simulink model "My_gfm_battery_sil"  (R2018b)
settings: Solver=ode45  StartTime=0.0  StopTime=100  MaxStep=1e-4  RelTol=1e-3
PreLoadFcn:
  | modelDir = fileparts(get_param(bdroot,'FileName'));
  | 
  | load_system(fullfile(modelDir,'controls_element_lib.slx'));
  | load_system(fullfile(modelDir,'test_sequence_lib.slx'));
InitFcn:
  | close all;
  | clear all;
  | clc;
  | 
  | % frequency nominals
  | F_NOM = 60;
  | W_NOM = 2 * pi * F_NOM;
  | 
  | % base values relative to inverter
  | % --------------------------------
  | VLL_INV_NOM = 480;
  | P_INV_NOM = 1e6;
  | Q_INV_NOM = 0.5e6;
  | S_INV_NOM = sqrt(P_INV_NOM^2 + Q_INV_NOM^2);
  | 
  | I_INV_BASE = S_INV_NOM/(sqrt(3)*VLL_INV_NOM);
  | Z_INV_BASE = VLL_INV_NOM^2/S_INV_NOM;
  | L_INV_BASE = Z_INV_BASE / W_NOM;
  | C_INV_BASE = 1 / (Z_INV_BASE * W_NOM);
  | 
  | % nominal ratings for power system model
  | % --------------------------------------
  | INVERTER_COUNT = 100;
  | 
  | VLV_NOM = VLL_INV_NOM;
  | VMV_NOM = 35e3;
  | VHV_NOM = 230e3;
  | S_PLANT = INVERTER_COUNT * S_INV_NOM;
  | 
  | N_GSU = VHV_NOM/VMV_NOM;
  | N_MVT = VMV_NOM/VLV_NOM;
  | 
  | I_LV_BASE = S_PLANT/(sqrt(3)*VLV_NOM);
  | I_MV_BASE = S_PLANT/(sqrt(3)*VMV_NOM);
  | I_HV_BASE = S_PLANT/(sqrt(3)*VHV_NOM);
  | 
  | Z_LV_BASE = VLV_NOM^2/S_PLANT;
  | Z_MV_BASE = VMV_NOM^2/S_PLANT;
  | Z_HV_BASE = VHV_NOM^2/S_PLANT;
  | 
  | L_LV_BASE = Z_LV_BASE / W_NOM;
  | L_MV_BASE = Z_MV_BASE / W_NOM;
  | L_HV_BASE = Z_HV_BASE / W_NOM;
  | C_LV_BASE = 1 / (Z_LV_BASE * W_NOM);
  | C_MV_BASE = 1 / (Z_MV_BASE * W_NOM);
  | C_HV_BASE = 1 / (Z_HV_BASE * W_NOM);
undefined symbols (not defined in the file): FreqFF_Sel, j
libraries: simulink x80, controls_element_lib x20, test_sequence_lib x16
(part 1 of 5)
settings Model: SimulationMode=accelerator  Creator=HussamAlatrash  LastModifiedBy=ahhei
settings DataIOCC: ReturnWorkspaceOutputs=on
settings OptimizationCC: EfficientMapNaN2IntZero=off
settings DebuggingCC: UnconnectedInputMsg=none  UnconnectedOutputMsg=none  UnconnectedLineMsg=none
settings HardwareCC: TargetBitPerPointer=64  TargetBitPerSizeT=64  TargetBitPerPtrDiffT=64  TargetLongLongMode=on  TargetIntDivRoundTo=Zero  TargetEndianess=LittleEndian  TargetWordSize=64  TargetHWDeviceType=MATLAB Host  ProdEqTarget=off
settings ModelReferenceCC: EnableRefExpFcnMdlSchedulingChecks=off
settings CodeAppCC: MaxIdLength=128
settings GRTTargetCC: TargetLangStandard=C89/C90 (ANSI)  CombineOutputUpdateFcns=off  GRTInterface=on

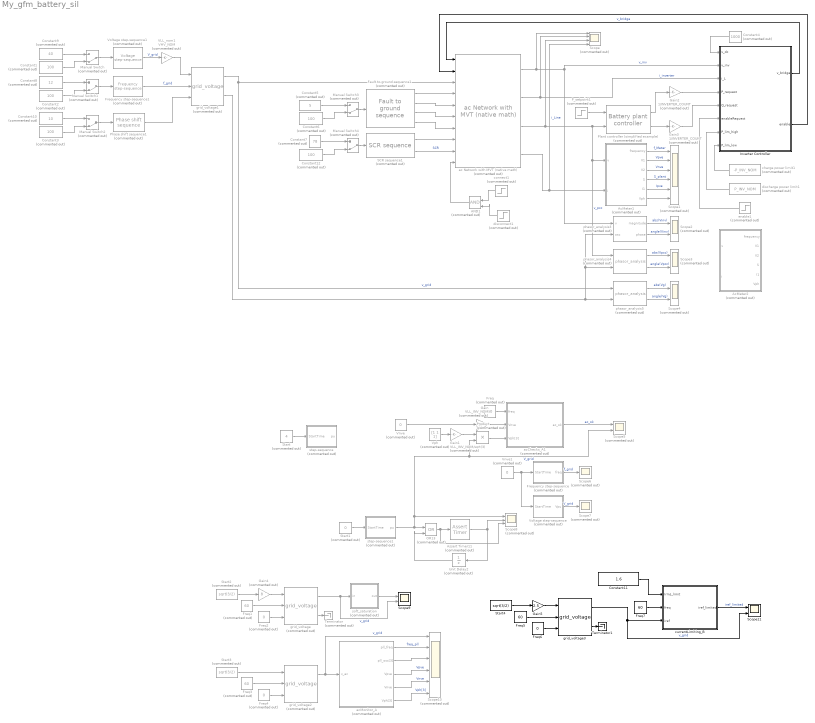
== system My_gfm_battery_sil ==
  AND1 : Logic  Commented=on  IconShape=distinctive  AllPortsSameDT=off  OutDataTypeStr=boolean
  AcMeter1 : Subsystem  Commented=on  AncestorBlock=test_sequence_lib/AcMeter  mask{VllRated=VHV_NOM}
      mask prompts: VllRated "Rated line voltage"
  AcMeter2 : Subsystem  Commented=on  AncestorBlock=test_sequence_lib/AcMeter  mask{VllRated=VHV_NOM}
      mask prompts: VllRated "Rated line voltage"
  Assert Timer11 : controls_element_lib/acChecks_A/Assert Timer  Commented=on  T_STEP=1e-3  TIMEOUT=2
  Constant{1..3,6,12} (5 alike) : Constant  Commented=on  Value=100
  Constant10 : Constant  Commented=on  Value=10
  Constant11 : Constant  Value=1.6
  Constant4 : Constant  Commented=on  Value=1000
  Constant5 : Constant  Commented=on  Value=5
  Constant7 : Constant  Commented=on  Value=78
  Constant8 : Constant  Commented=on  Value=12
  Constant9 : Constant  Commented=on  Value=40
  Fault to ground sequence1 : test_sequence_lib/Fault to ground sequence  Commented=on  SystemSampleTime=-1
  Freq : Constant  Commented=on  Value=60
  Freq1 : Constant  Commented=on  Value=60
  Freq2 : Constant  Commented=on  Value=0
  Freq3 : Constant  Commented=on  Value=60
  Freq4 : Constant  Commented=on  Value=0
  Freq5 : Constant  Value=60
  Freq6 : Constant  Value=0
  Freq7 : Constant  Value=60
  Frequency step-sequence : Subsystem  Commented=on  AncestorBlock=test_sequence_lib/Frequency step-sequence
  Frequency step-sequence1 : test_sequence_lib/Frequency step-sequence  Commented=on  SystemSampleTime=-1
  Gain : Gain  Commented=on  Gain=VLL_INV_NOM
  Gain1 : Gain  Commented=on  Gain=VLL_INV_NOM/sqrt(3)
  Gain2 : Gain  Commented=on  Gain=1/INVERTER_COUNT
  Gain3 : Gain  Commented=on  Gain=1/INVERTER_COUNT
  Gain4 : Gain  Commented=on  Gain=8
  Gain5 : Gain  Gain=2.5
  Inverter Controller : Subsystem
  Manual Switch{,1..4} (5 alike) : ManualSwitch  Commented=on  CurrentSetting=0
  OR13 : Logic  Commented=on  Operator=OR  IconShape=distinctive  AllPortsSameDT=off  OutDataTypeStr=boolean
  P_setpoint1 : Step  Commented=on  Time=4  After=S_PLANT*0.5  SampleTime=0
  Phase shift sequence1 : test_sequence_lib/Phase shift sequence  Commented=on  SystemSampleTime=-1
  Plant controller (simplified example) : controls_element_lib/Battery plant controller  Commented=on  SystemSampleTime=-1
  Product : Product  Commented=on
  SCR sequence1 : test_sequence_lib/SCR sequence  Commented=on  SystemSampleTime=-1
  Scope : Scope  Commented=on  NumInputPorts=4
  Scope1 : Scope  Commented=on  NumInputPorts=6
  Scope10 : Scope  Commented=on  NumInputPorts=6
  Scope11 : Scope  NumInputPorts=2
  Scope{2..5} (4 alike) : Scope  Commented=on  NumInputPorts=2
  Scope6 : Scope  Commented=on
  Scope7 : Scope  Commented=on
  Scope8 : Scope  Commented=on  NumInputPorts=3
  Scope9 : Scope  NumInputPorts=2
  Start : Constant  Commented=on  Value=4
  Start1 : Constant  Commented=on  Value=0
  Start2 : Constant  Commented=on  Value=sqrt(3/2)
  Start3 : Constant  Commented=on  Value=sqrt(3/2)
  Start4 : Constant  Value=sqrt(3/2)
  Terminator : Terminator  Commented=on
  Terminator1 : Terminator
  Unit Delay2 : UnitDelay  Commented=on  SampleTime=-1
  VLL_nom1 : Gain  Commented=on  Gain=VHV_NOM
  Vnve : Constant  Commented=on  Value=0
  Vnve1 : Constant  Commented=on  Value=0
  Voltage step-sequence : Subsystem  Commented=on  AncestorBlock=test_sequence_lib/Voltage step-sequence
  Voltage step-sequence1 : test_sequence_lib/Voltage step-sequence  Commented=on  SystemSampleTime=-1
  Vph : Constant  Commented=on  Value=[1 1 1]
  ac Network with MVT (native math) : test_sequence_lib/ac Network with MVT (native math)  Commented=on  SystemSampleTime=-1
  acChecks_A1 : Subsystem  Commented=on  AncestorBlock=controls_element_lib/acChecks_A  mask{VllRated=VLL_INV_NOM, nominalFrequency=F_NOM, tRequalify=2, T_CNTL=1e-3}
      mask prompts: VllRated "Rated line-to-line voltage (V)"; nominalFrequency "Nominal line frequency (Hz)"; tRequalify "Reconnection time (sec)"; T_CNTL "Operating sample time"
  "acMonitor_A " : Subsystem  Commented=on  AncestorBlock=controls_element_lib/acMonitor_A  mask{VllRated=VLL_INV_NOM, nominalFrequency=F_NOM}
      mask prompts: VllRated "Rated line-to-line voltage (V)"; nominalFrequency "Nominal line frequency (Hz)"
  charge power limit1 : Constant  Commented=on  Value=-P_INV_NOM
  connect1 : Step  Commented=on  Time=0  SampleTime=0
  currentLimiting_B : Subsystem  AncestorBlock=controls_element_lib/currentLimiting_B  mask{IRated=1, peakSoftLimit=2.6, peakHardLimit=3.6}
      mask prompts: IRated "Rated current (A)"; peakSoftLimit "Soft peak limit (pu)"; peakHardLimit "Hard peak limit (pu)"
  discharge power limit1 : Constant  Commented=on  Value=P_INV_NOM
  disconnect1 : Step  Commented=on  Time=10  Before=1  After=0  SampleTime=0
  enable1 : Step  Commented=on  Time=0.5  SampleTime=0
  grid_voltage : test_sequence_lib/grid_voltage  Commented=on  SystemSampleTime=-1
  grid_voltage1 : test_sequence_lib/grid_voltage  Commented=on  SystemSampleTime=-1
  grid_voltage2 : test_sequence_lib/grid_voltage  Commented=on  SystemSampleTime=-1
  grid_voltage3 : test_sequence_lib/grid_voltage  SystemSampleTime=-1
  phasor_analysis3 : Subsystem  Commented=on  AncestorBlock=test_sequence_lib/phasor_analysis
  phasor_analysis4 : test_sequence_lib/phasor_analysis  Commented=on  SystemSampleTime=-1
  phasor_analysis5 : test_sequence_lib/phasor_analysis  Commented=on  SystemSampleTime=-1
  soft_saturation : Subsystem  Commented=on  mask{soft_limit=2.6*sqrt(2)*sqrt(1/2), hard_limit=3.6*sqrt(2)*sqrt(1/2), Xau=1}
      mask prompts: soft_limit "Soft limit"; hard_limit "Hard limit"; Xau "Saturation Rate"
  step-sequence : Subsystem  Commented=on  AncestorBlock=test_sequence_lib/Voltage step-sequence
  step-sequence1 : Subsystem  Commented=on  AncestorBlock=test_sequence_lib/Voltage step-sequence
  wires:
  Voltage step-sequence1/1 -> VLL_nom1/1  "V_grid"
  Manual Switch/1 -> Voltage step-sequence1/1
  Fault to ground sequence1/2 -> ac Network with MVT (native math)/5
  AND1/1 -> ac Network with MVT (native math)/10
  Constant4/1 -> Inverter Controller/1(v_dc)
  AcMeter1/3(V2) -> Scope1/3  "Vnve"
  discharge power limit1/1 -> Inverter Controller/7(P_lim_high)
  Fault to ground sequence1/3 -> ac Network with MVT (native math)/6
  AcMeter1/6(Vph) -> Scope1/6
  Inverter Controller/1(v_bridge) -> ac Network with MVT (native math)/1  "v_bridge"
  AcMeter1/2(V1) -> Scope1/2  "Vpve"
  Plant controller (simplified example)/1 -> Gain2/1
  ac Network with MVT (native math)/1 -> Inverter Controller/2(v_inv), phasor_analysis3/1(v), Scope/1  "v_inv"
  P_setpoint1/1 -> Plant controller (simplified example)/1
  phasor_analysis5/1 -> Scope4/1  "abs(Vg)"
  AcMeter1/5(I1) -> Scope1/5  "Ipve"
  Gain3/1 -> Inverter Controller/5(Q_request)
  Plant controller (simplified example)/2 -> Gain3/1
  grid_voltage1/1 -> ac Network with MVT (native math)/3, phasor_analysis5/1  "v_grid"
  SCR sequence1/1 -> ac Network with MVT (native math)/8
  phasor_analysis3/1(magnitude) -> Scope2/1  "abs(Vinv)"
  Phase shift sequence1/1 -> grid_voltage1/3
  AcMeter1/4(S) -> Scope1/4  "S_plant"
  ac Network with MVT (native math)/4 -> Scope/4, AcMeter1/2(i)  "i_Line"
  AcMeter1/1(frequency) -> Scope1/1  "f_Meter"
  VLL_nom1/1 -> grid_voltage1/1
  phasor_analysis3/2(phase) -> Scope2/2  "angle(Vinv)"
  SCR sequence1/2 -> ac Network with MVT (native math)/9  "SCR"
  ac Network with MVT (native math)/2 -> Inverter Controller/3(i_L), Scope/2  "i_inverter"
  disconnect1/1 -> AND1/2
  Fault to ground sequence1/4 -> ac Network with MVT (native math)/7
  Gain2/1 -> Inverter Controller/4(P_request)
  ac Network with MVT (native math)/3 -> Plant controller (simplified example)/2, phasor_analysis4/1, AcMeter1/1(v), Scope/3  "v_pcc"
  charge power limit1/1 -> Inverter Controller/8(P_lim_low)
  Inverter Controller/2(enable) -> ac Network with MVT (native math)/2
  Frequency step-sequence1/1 -> grid_voltage1/2  "f_grid"
  Fault to ground sequence1/1 -> ac Network with MVT (native math)/4
  grid_voltage1/2 -> phasor_analysis4/2, phasor_analysis3/2(osc), phasor_analysis5/2
  phasor_analysis5/2 -> Scope4/2  "angle(Vg)"
  enable1/1 -> Inverter Controller/6(enableRequest)
  connect1/1 -> AND1/1
  Constant9/1 -> Manual Switch/1
  Constant1/1 -> Manual Switch/2
  Constant2/1 -> Manual Switch1/2
  Manual Switch1/1 -> Frequency step-sequence1/1
  Constant8/1 -> Manual Switch1/1
  Manual Switch2/1 -> Phase shift sequence1/1
  Constant3/1 -> Manual Switch2/2
  Constant10/1 -> Manual Switch2/1
  Constant6/1 -> Manual Switch3/2
  Constant5/1 -> Manual Switch3/1
  Manual Switch3/1 -> Fault to ground sequence1/1
  Constant7/1 -> Manual Switch4/1
  Constant12/1 -> Manual Switch4/2
  Manual Switch4/1 -> SCR sequence1/1
  phasor_analysis4/1 -> Scope3/1  "abs(Vpcc)"
  phasor_analysis4/2 -> Scope3/2  "angle(Vpcc)"
  Vnve/1 -> Gain/1
  Freq/1 -> acChecks_A1/1(freq)
  Vph/1 -> Gain1/1
  acChecks_A1/1(ac_ok) -> Scope5/1  "ac_ok"
  Gain/1 -> acChecks_A1/2(Vnve)
  Vnve1/1 -> Voltage step-sequence/1(StartTime), Frequency step-sequence/1(StartTime)
  Frequency step-sequence/1(freq) -> Scope6/1  "f_grid"
  Voltage step-sequence/1(Vpu) -> Scope7/1  "V_grid"
  Start/1 -> step-sequence/1(StartTime)
  Gain1/1 -> Product/1
  Product/1 -> acChecks_A1/3(Vph[3])
  step-sequence1/1(pu) -> Scope5/2, Product/2, Scope8/1, OR13/1  "V_grid"
  OR13/1 -> Scope8/3, Assert Timer11/1
  Unit Delay2/1 -> OR13/2
  Start1/1 -> step-sequence1/1(StartTime)
  Assert Timer11/1 -> Scope8/2, Unit Delay2/1
  grid_voltage/1 -> Scope9/2, soft_saturation/1(in)  "v_grid"
  Start2/1 -> Gain4/1
  Gain4/1 -> grid_voltage/1
  Freq1/1 -> grid_voltage/2
  Freq2/1 -> grid_voltage/3
  soft_saturation/1(out) -> Scope9/1
  grid_voltage/2 -> Terminator/1
  Freq4/1 -> grid_voltage2/3
  Freq3/1 -> grid_voltage2/2
  Start3/1 -> grid_voltage2/1
  grid_voltage2/1 -> Scope10/1, "acMonitor_A "/1(v_ac)  "v_grid"
  "acMonitor_A "/1(pll_freq) -> Scope10/2  "freq_pll"
  "acMonitor_A "/2(pll_osc[3]) -> Scope10/3
  "acMonitor_A "/3(Vpve) -> Scope10/4  "Vpve"
  "acMonitor_A "/4(Vnve) -> Scope10/5  "Vnve"
  "acMonitor_A "/5(Vph[3]) -> Scope10/6  "Vph[3]"
  Constant11/1 -> currentLimiting_B/1(Irms_limit)
  Start4/1 -> Gain5/1
  Freq6/1 -> grid_voltage3/3
  Gain5/1 -> grid_voltage3/1
  Freq5/1 -> grid_voltage3/2
  grid_voltage3/2 -> Terminator1/1
  grid_voltage3/1 -> Scope11/2, currentLimiting_B/3(iref)  "v_grid"
  Freq7/1 -> currentLimiting_B/2(freq)
  currentLimiting_B/1(iref_limited) -> Scope11/1  "iref_limited"

== system My_gfm_battery_sil/AcMeter1 ==
  v : Inport
  i : Inport  Port=2
  Conj : Math  Operator=conj  SaturateOnIntegerOverflow=on
  PLL_3ph : Subsystem
  Product : Product
  RMS calculator : Subsystem
  Scope : Scope  NumInputPorts=3
  Scope1 : Scope  NumInputPorts=4
  Sum of Elements : Sum  Commented=through  Inputs=+
  overVnom : Gain  Gain=1/VllRated
  phasor_analysis : Subsystem
  phasor_analysis1 : Subsystem  AncestorBlock=test_sequence_lib/AcMeter/phasor_analysis
  sqrt(3) : Gain  Gain=sqrt(3)
  sqrt(3)1 : Gain  Gain=sqrt(3)
  frequency : Outport  VectorParamsAs1DForOutWhenUnconnected=on
  V1 : Outport  Port=2  VectorParamsAs1DForOutWhenUnconnected=on
  V2 : Outport  Port=3  VectorParamsAs1DForOutWhenUnconnected=on
  S : Outport  Port=4  VectorParamsAs1DForOutWhenUnconnected=on
  I1 : Outport  Port=5  VectorParamsAs1DForOutWhenUnconnected=on
  Vph : Outport  Port=6  VectorParamsAs1DForOutWhenUnconnected=on
  wires:
  RMS calculator/1(out[3]) -> Vph/1
  PLL_3ph/2(osc[3]) -> phasor_analysis/2(osc), phasor_analysis1/2(osc)
  phasor_analysis/1(perPh) -> Scope/1
  Sum of Elements/1 -> Scope1/4, S/1  "S"
  v/1 -> RMS calculator/1(in[3]), phasor_analysis/1(in), overVnom/1
  PLL_3ph/1(freq) -> frequency/1
  overVnom/1 -> PLL_3ph/1(ref)
  Conj/1 -> Scope1/2, Product/2
  Product/1 -> Scope1/3, Sum of Elements/1
  phasor_analysis/2(pve) -> Scope/2, Scope1/1, Product/1, sqrt(3)/1  "Vpve_LN"
  phasor_analysis/3(nve) -> Scope/3, sqrt(3)1/1
  phasor_analysis1/2(pve) -> I1/1, Conj/1  "Ipve"
  sqrt(3)1/1 -> V2/1  "Vnve_LL"
  i/1 -> phasor_analysis1/1(in)
  sqrt(3)/1 -> V1/1  "Vpve_LL"

== system My_gfm_battery_sil/AcMeter2 ==
  v : Inport
  i : Inport  Port=2
  Conj : Math  Operator=conj  SaturateOnIntegerOverflow=on
  PLL_3ph : Subsystem
  Product : Product
  RMS calculator : Subsystem
  Scope : Scope  NumInputPorts=3
  Scope1 : Scope  NumInputPorts=4
  Sum of Elements : Sum  Inputs=+
  overVnom : Gain  Gain=1/VllRated
  phasor_analysis : Subsystem
  phasor_analysis1 : Subsystem  AncestorBlock=test_sequence_lib/AcMeter/phasor_analysis
  sqrt(3) : Gain  Gain=sqrt(3)
  sqrt(3)1 : Gain  Gain=sqrt(3)
  frequency : Outport  VectorParamsAs1DForOutWhenUnconnected=on
  V1 : Outport  Port=2  VectorParamsAs1DForOutWhenUnconnected=on
  V2 : Outport  Port=3  VectorParamsAs1DForOutWhenUnconnected=on
  S : Outport  Port=4  VectorParamsAs1DForOutWhenUnconnected=on
  I1 : Outport  Port=5  VectorParamsAs1DForOutWhenUnconnected=on
  Vph : Outport  Port=6  VectorParamsAs1DForOutWhenUnconnected=on
  wires:
  RMS calculator/1(out[3]) -> Vph/1
  PLL_3ph/2(osc[3]) -> phasor_analysis/2(osc), phasor_analysis1/2(osc)
  phasor_analysis/1(perPh) -> Scope/1, Product/1, Scope1/1
  Sum of Elements/1 -> Scope1/4, S/1  "S"
  v/1 -> RMS calculator/1(in[3]), phasor_analysis/1(in), overVnom/1
  PLL_3ph/1(freq) -> frequency/1
  phasor_analysis1/1(perPh) -> Conj/1
  overVnom/1 -> PLL_3ph/1(ref)
  Conj/1 -> Scope1/2, Product/2
  Product/1 -> Scope1/3, Sum of Elements/1
  phasor_analysis/2(pve) -> Scope/2, sqrt(3)/1  "Vpve_LN"
  phasor_analysis/3(nve) -> Scope/3, sqrt(3)1/1
  phasor_analysis1/2(pve) -> I1/1  "Ipve"
  sqrt(3)1/1 -> V2/1  "Vnve_LL"
  i/1 -> phasor_analysis1/1(in)
  sqrt(3)/1 -> V1/1  "Vpve_LL"

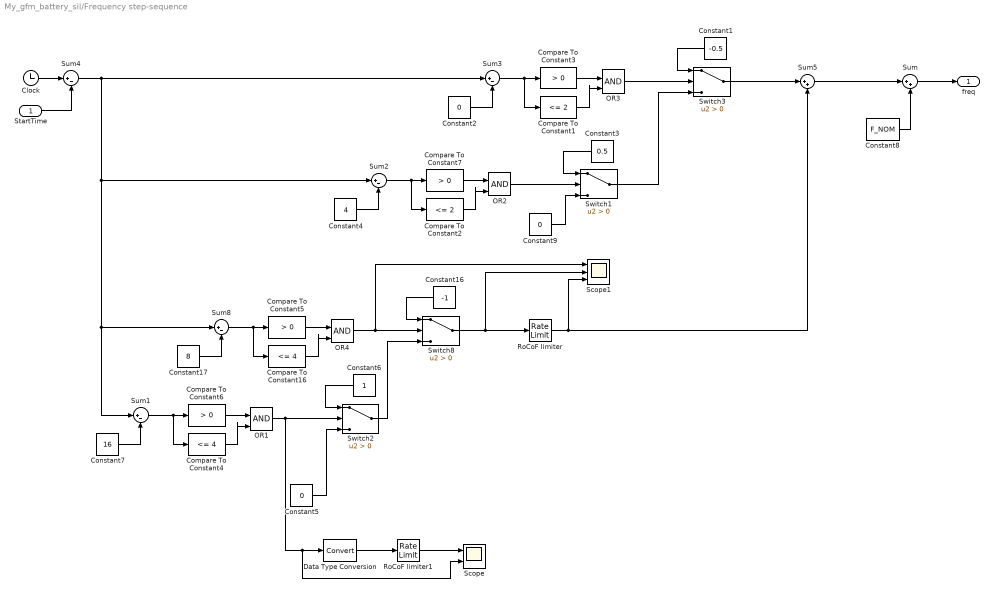
== system My_gfm_battery_sil/Frequency step-sequence ==
  StartTime : Inport
  Clock : Clock
  Compare To Constant1 : simulink/Logic and Bit Operations/Compare To Constant  relop=<=  const=2  OutDataTypeStr=boolean
  Compare To Constant16 : simulink/Logic and Bit Operations/Compare To Constant  relop=<=  const=4  OutDataTypeStr=boolean
  Compare To Constant2 : simulink/Logic and Bit Operations/Compare To Constant  relop=<=  const=2  OutDataTypeStr=boolean
  Compare To Constant{3,5..7} (4 alike) : simulink/Logic and Bit Operations/Compare To Constant  relop=>  const=0  OutDataTypeStr=boolean
  Compare To Constant4 : simulink/Logic and Bit Operations/Compare To Constant  relop=<=  const=4  OutDataTypeStr=boolean
  Constant1 : Constant  Value=-0.5
  Constant16 : Constant  Value=-1
  Constant17 : Constant  Value=8
  Constant2 : Constant  Value=0
  Constant3 : Constant  Value=0.5
  Constant4 : Constant  Value=4
  Constant5 : Constant  Value=0
  Constant6 : Constant
  Constant7 : Constant  Value=16
  Constant8 : Constant  Value=F_NOM
  Constant9 : Constant  Value=0
  Data Type Conversion : DataTypeConversion
  OR{1..4} (4 alike) : Logic  IconShape=distinctive  AllPortsSameDT=off  OutDataTypeStr=boolean
  RoCoF limiter : RateLimiter  SampleTimeMode=inherited
  RoCoF limiter1 : RateLimiter  SampleTimeMode=inherited
  Scope : Scope  NumInputPorts=2
  Scope1 : Scope  NumInputPorts=3
  Sum : Sum  Inputs=|++
  Sum{1..4,8} (5 alike) : Sum  Inputs=|+-
  Sum5 : Sum  Inputs=|++
  Switch{1..3,8} (4 alike) : Switch  Criteria=u2 > Threshold
  freq : Outport  VectorParamsAs1DForOutWhenUnconnected=on
  wires:
  Switch2/1 -> Switch8/3
  Constant16/1 -> Switch8/1
  OR4/1 -> Scope1/1, Switch8/2
  Compare To Constant5/1 -> OR4/1
  Sum8/1 -> Compare To Constant5/1, Compare To Constant16/1
  Constant17/1 -> Sum8/2
  Compare To Constant16/1 -> OR4/2
  Constant5/1 -> Switch2/3
  Constant6/1 -> Switch2/1
  OR1/1 -> Scope/2, Data Type Conversion/1, Switch2/2
  Compare To Constant6/1 -> OR1/1
  Sum1/1 -> Compare To Constant6/1, Compare To Constant4/1
  Constant7/1 -> Sum1/2
  Compare To Constant4/1 -> OR1/2
  Compare To Constant2/1 -> OR2/2
  Constant4/1 -> Sum2/2
  Sum2/1 -> Compare To Constant2/1, Compare To Constant7/1
  Compare To Constant7/1 -> OR2/1
  OR2/1 -> Switch1/2
  Constant3/1 -> Switch1/1
  Compare To Constant1/1 -> OR3/2
  Constant2/1 -> Sum3/2
  Sum3/1 -> Compare To Constant1/1, Compare To Constant3/1
  Compare To Constant3/1 -> OR3/1
  OR3/1 -> Switch3/2
  Constant1/1 -> Switch3/1
  Sum4/1 -> Sum3/1, Sum2/1, Sum8/1, Sum1/1
  Switch1/1 -> Switch3/3
  Clock/1 -> Sum4/1
  StartTime/1 -> Sum4/2
  Switch8/1 -> Scope1/2, RoCoF limiter/1
  Sum/1 -> freq/1
  Constant8/1 -> Sum/2
  Sum5/1 -> Sum/1
  RoCoF limiter/1 -> Scope1/3, Sum5/2
  Constant9/1 -> Switch1/3
  RoCoF limiter1/1 -> Scope/1
  Data Type Conversion/1 -> RoCoF limiter1/1
  Switch3/1 -> Sum5/1

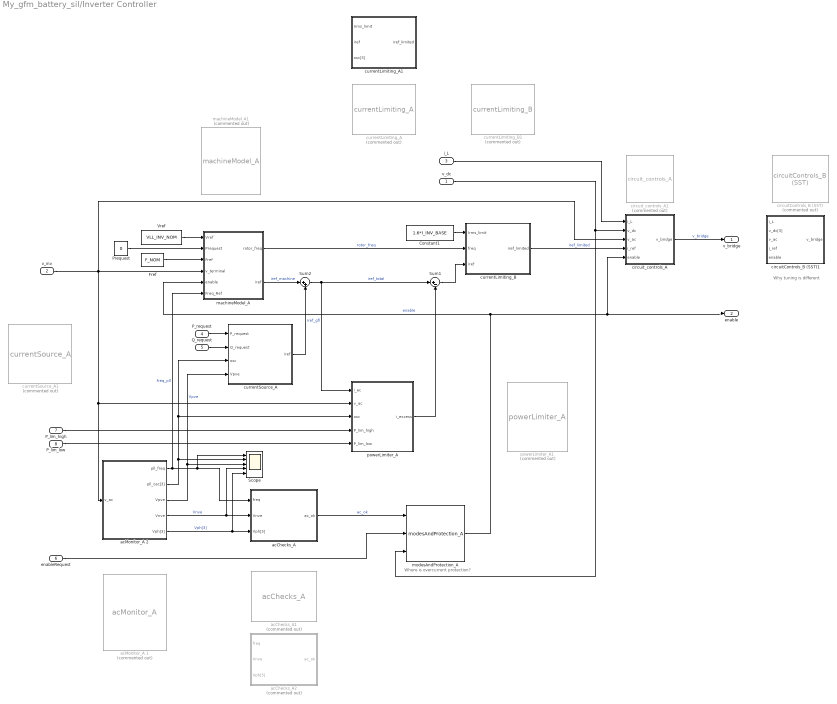
== system My_gfm_battery_sil/Inverter Controller ==
  note: Why tuning is different
  note: Where is overcurrent protection?
  v_dc : Inport
  v_inv : Inport  Port=2
  i_L : Inport  Port=3
  P_request : Inport  Port=4
  Q_request : Inport  Port=5
  enableRequest : Inport  Port=6
  P_lim_high : Inport  Port=7
  P_lim_low : Inport  Port=8
  Constant1 : Constant  Value=1.6*I_INV_BASE
  Fref : Constant  Value=F_NOM
  Prequest : Constant  Value=0
  Scope : Scope  NumInputPorts=5
  Sum1 : Sum  Inputs=|+-
  Sum2 : Sum  Inputs=|++
  Vref : Constant  Value=VLL_INV_NOM
  acChecks_A : Subsystem  AncestorBlock=controls_element_lib/acChecks_A  mask{VllRated=VLL_INV_NOM, nominalFrequency=F_NOM, tRequalify=2, T_CNTL=1e-3}
      mask prompts: VllRated "Rated line-to-line voltage (V)"; nominalFrequency "Nominal line frequency (Hz)"; tRequalify "Reconnection time (sec)"; T_CNTL "Operating sample time"
  acChecks_A1 : controls_element_lib/acChecks_A  Commented=on  VllRated=VLL_INV_NOM  nominalFrequency=F_NOM  tRequalify=2  T_CNTL=1e-3
  acChecks_A2 : Subsystem  Commented=on  AncestorBlock=controls_element_lib/acChecks_A  mask{VllRated=VLL_INV_NOM, NominalFrequency=F_NOM, Ts=1e-3, Time1=2, Time2=0, VHi=0, VLo=0, FHi=0, FLo=0, VNeg=0, Time3=0, OV1=0, OV1_Time=0, OV2=0, OV2_Time=0, OV3=0, OV3_Time=0, UV1=0, UV1_Time=0, UV2=0, UV2_Time=0, UV3=0, UV3_Time=0, OF1=0, OF1_Time=0, OF2=0, OF2_Time=0, OF3=0, OF3_Time=0, UF1=0, UF1_Time=0, UF2=0, UF2_Time=0, UF3=0, UF3_Time=0}
      mask prompts: VllRated "Rated Line-to-Line Voltage (V)"; NominalFrequency "Nominal Line Frequency (Hz)"; Ts "Operating Sample Time (sec)"; Time1 "Reconnection Time (sec)"; Time2 "Connect Out-of-Condition Delay (sec)"; VHi "High Voltage Threshold (pu)"; VLo "Low Voltage Threshold (pu)"; FHi "High Frequency Threshold (Hz)"; FLo "Low Frequency Threshold (Hz)"; VNeg "Negative Sequence Voltage Threshold (pu)"; Time3 "Trip Out-of-Condition Delay (sec)"; OV1 "OV PickUp 1 (pu)"; OV1_Time "OV Time 1 (sec)"; OV2 "OV PickUp 2 (pu)"; OV2_Time "OV Time 2 (sec)"; OV3 "OV PickUp 3 (pu)"; OV3_Time "OV Time 3 (sec)"; UV1 "UV PickUp 1 (pu)"; UV1_Time "UV Time 1 (sec)"; UV2 "UV PickUp 2 (pu)"; UV2_Time "UV Time 2 (sec)"; UV3 "UV PickUp 3 (pu)"; UV3_Time "UV Time 3 (sec)"; OF1 "OF PickUp 1 (Hz)"; OF1_Time "OF Time 1 (pu)"; OF2 "OF PickUp 2 (Hz)"; OF2_Time "OF Time 2 (pu)"; OF3 "OF PickUp 3 (Hz)"; OF3_Time "OF Time 3 (pu)"; UF1 "UF PickUp 1 (Hz)"; UF1_Time "UF Time 1 (sec)"; UF2 "UF PickUp 2 (Hz)"; UF2_Time "UF Time 2 (sec)"; UF3 "UF PickUp 3 (Hz)"; UF3_Time "UF Time 3 (sec)"
      mask DialogControl DescGroupVar Prompt: ACChecks
      mask DialogControl DecsTextVar Prompt: Grid Checks for Connection and Tripping
      mask DialogControl ParameterGroupVar Prompt: General Parameters
      mask DialogControl Container11 Prompt: Connect Settings
      mask DialogControl Container20 Prompt: Thresholds
      mask DialogControl Container3 Prompt: Trip Settings
      mask DialogControl Container12 Prompt: General Parameters
      mask DialogControl Container15 Prompt: Over Voltage Settings
      mask DialogControl Container4 Prompt: Over Voltage
      mask DialogControl Container19 Prompt: Under Voltage Settings
      mask DialogControl Container7 Prompt: Under Voltage
      mask DialogControl Container17 Prompt: Over Frequency Settings
      mask DialogControl Container9 Prompt: Over Frequency
      mask DialogControl Container16 Prompt: Under Frequency Settings
      mask DialogControl Container10 Prompt: Under Frequency
  acMonitor_A 1 : controls_element_lib/acMonitor_A  Commented=on  VllRated=VLL_INV_NOM  nominalFrequency=F_NOM
  acMonitor_A 2 : Subsystem  AncestorBlock=controls_element_lib/acMonitor_A  mask{VllRated=VLL_INV_NOM, nominalFrequency=F_NOM}
      mask prompts: VllRated "Rated line-to-line voltage (V)"; nominalFrequency "Nominal line frequency (Hz)"
  circuitControls_B (SST) : controls_element_lib/circuitControls_B (SST)  Commented=on  SystemSampleTime=-1
  circuitControls_B (SST)1 : Subsystem  AncestorBlock=controls_element_lib/circuitControls_B (SST)
  circuit_controls_A : Subsystem  AncestorBlock=controls_element_lib/circuit_controls_A
  circuit_controls_A1 : controls_element_lib/circuit_controls_A  Commented=on  SystemSampleTime=-1
  currentLimiting_A : controls_element_lib/currentLimiting_A  Commented=on  IRated=I_INV_BASE  peakSoftLimit=2.6  peakHardLimit=3.6
  currentLimiting_A1 : Subsystem  AncestorBlock=controls_element_lib/currentLimiting_A  mask{IRated=I_INV_BASE, peakSoftLimit=2.6, peakHardLimit=3.6}
      mask prompts: IRated "Rated current (A)"; peakSoftLimit "Soft peak limit (pu)"; peakHardLimit "Hard peak limit (pu)"
  currentLimiting_B : Subsystem  AncestorBlock=controls_element_lib/currentLimiting_B  mask{IRated=1, peakSoftLimit=2.6, peakHardLimit=3.6}
      mask prompts: IRated "Rated current (A)"; peakSoftLimit "Soft peak limit (pu)"; peakHardLimit "Hard peak limit (pu)"
  currentLimiting_B1 : controls_element_lib/currentLimiting_B  Commented=on  IRated=I_INV_BASE  peakSoftLimit=2.6  peakHardLimit=3.6
  currentSource_A : Subsystem  AncestorBlock=controls_element_lib/currentSource_A  mask{VllRated=VLL_INV_NOM, SRated=S_INV_NOM, nominalFrequency=F_NOM, Plimit=P_INV_NOM/S_INV_NOM, Qlimit=Q_INV_NOM/S_INV_NOM}
      mask prompts: VllRated "Rated line-to-line voltage (V)"; SRated "Rated power (VA)"; nominalFrequency "Nominal line frequency (Hz)"; Plimit "Real power request limit (pu)"; Qlimit "Reactive power request limit (pu)"
  currentSource_A1 : controls_element_lib/currentSource_A  Commented=on  VllRated=VLL_INV_NOM  SRated=S_INV_NOM  nominalFrequency=F_NOM  Plimit=P_INV_NOM/S_INV_NOM  Qlimit=Q_INV_NOM/S_INV_NOM
  machineModel_A : Subsystem  AncestorBlock=controls_element_lib/machineModel_A  mask{SRated=S_INV_NOM, VllRated=VLL_INV_NOM, nominalFrequency=F_NOM, inertialConstant=2.5, kDroop=1, kDamper=2, Xs=0.3, rs=0.08, Qlimit=0.5, wExciter=10}
      mask prompts: SRated "Rated power (VA)"; VllRated "Rated Voltage (Volts, line-to-line)"; nominalFrequency "Nominal frequency (Hz)"; inertialConstant "Inertial constant (seconds)"; kDroop "Droop gain (pu/Hz)"; kDamper "Damper gain (pu/Hz)"; Xs "Stator reactance (pu)"; rs "Stator resistance (pu)"; Qlimit "Reactive power request limit (pu)"; wExciter "Exciter Bandwidth (rad)"
  machineModel_A1 : controls_element_lib/machineModel_A  Commented=on  SRated=S_INV_NOM  VllRated=VLL_INV_NOM  nominalFrequency=F_NOM  inertialConstant=2.5  kDroop=1  kDamper=2  Xs=0.3  rs=0.08  Qlimit=0.5  wExciter=10
  modesAndProtection_A : controls_element_lib/modesAndProtection_A  dcOvervotlageThreshold=1800  dcUndervotlageThreshold=700  dcTripClearTimeout=0.2
  powerLimiter_A : Subsystem  AncestorBlock=controls_element_lib/powerLimiter_A  mask{VllRated=VLL_INV_NOM, nominalFrequency=F_NOM, wPowerLimiter=3}
      mask prompts: VllRated "Rated line-to-line voltage (V)"; nominalFrequency "Nominal line frequency (Hz)"; wPowerLimiter "Bandwidth (rad)"
  powerLimiter_A1 : controls_element_lib/powerLimiter_A  Commented=on  VllRated=VLL_INV_NOM  nominalFrequency=F_NOM  wPowerLimiter=3
  v_bridge : Outport  VectorParamsAs1DForOutWhenUnconnected=on
  enable : Outport  Port=2  VectorParamsAs1DForOutWhenUnconnected=on
  wires:
  Vref/1 -> machineModel_A/1(Vref)
  Prequest/1 -> machineModel_A/2(Prequest)
  Fref/1 -> machineModel_A/3(Fref)
  machineModel_A/2(iref) -> Sum2/1  "iref_machine"
  acMonitor_A 2/2(pll_osc[3]) -> Scope/2, currentSource_A/3(osc), powerLimiter_A/3(osc)
  currentLimiting_B/1(iref_limited) -> circuit_controls_A/4(i_ref)  "iref_limited"
  currentSource_A/1(iref) -> Sum2/2  "iref_gfl"
  Sum2/1 -> Sum1/1, powerLimiter_A/1(i_ac)  "iref_total"
  acMonitor_A 2/3(Vpve) -> Scope/3, currentSource_A/4(Vpve)  "Vpve"
  Q_request/1 -> currentSource_A/2(Q_request)
  P_request/1 -> currentSource_A/1(P_request)
  enableRequest/1 -> modesAndProtection_A/2
  modesAndProtection_A/1 -> machineModel_A/5(enable), circuit_controls_A/5(enable), enable/1  "enable"
  acMonitor_A 2/5(Vph[3]) -> Scope/5, acChecks_A/3(Vph[3])  "Vph[3]"
  acChecks_A/1(ac_ok) -> modesAndProtection_A/1  "ac_ok"
  Constant1/1 -> currentLimiting_B/1(Irms_limit)
  acMonitor_A 2/1(pll_freq) -> Scope/1, acChecks_A/1(freq), machineModel_A/6(Freq_Ref)  "freq_pll"
  acMonitor_A 2/4(Vnve) -> Scope/4, acChecks_A/2(Vnve)  "Vnve"
  P_lim_low/1 -> powerLimiter_A/5(P_lim_low)
  P_lim_high/1 -> powerLimiter_A/4(P_lim_high)
  powerLimiter_A/1(i_excess) -> Sum1/2
  Sum1/1 -> currentLimiting_B/3(iref)
  v_dc/1 -> circuit_controls_A/2(v_dc), modesAndProtection_A/3
  circuit_controls_A/1(v_bridge) -> v_bridge/1  "v_bridge"
  machineModel_A/1(rotor_freq) -> currentLimiting_B/2(freq)  "rotor_freq"
  i_L/1 -> circuit_controls_A/1(i_L)
  v_inv/1 -> acMonitor_A 2/1(v_ac), powerLimiter_A/2(v_ac), machineModel_A/4(v_terminal), circuit_controls_A/3(v_ac)

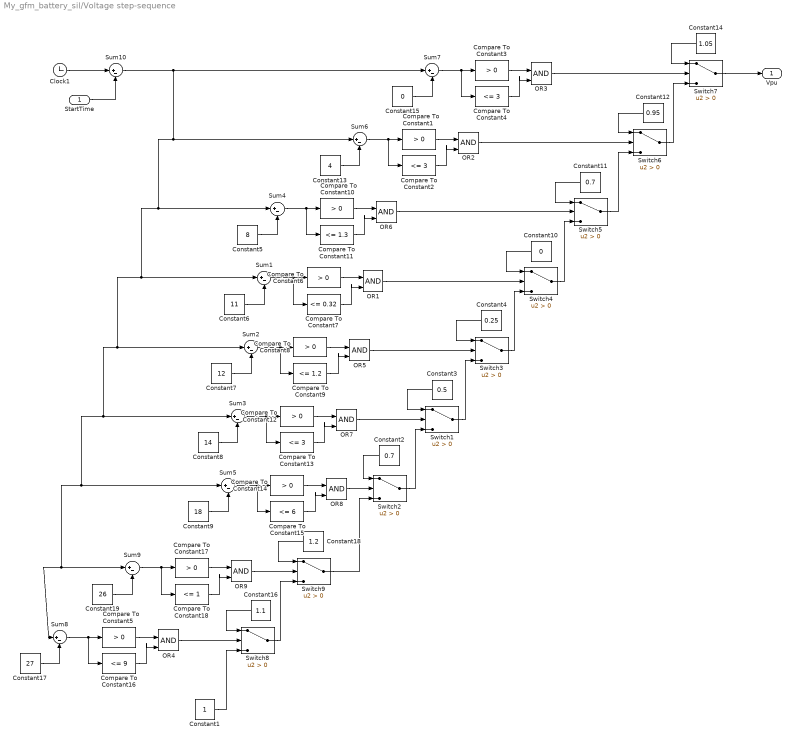
== system My_gfm_battery_sil/Voltage step-sequence ==
  StartTime : Inport
  Clock1 : Clock
  Compare To Constant{1,3,5..6,8,10,12,14,17} (9 alike) : simulink/Logic and Bit Operations/Compare To Constant  relop=>  const=0  OutDataTypeStr=boolean
  Compare To Constant11 : simulink/Logic and Bit Operations/Compare To Constant  relop=<=  const=1.3  OutDataTypeStr=boolean
  Compare To Constant13 : simulink/Logic and Bit Operations/Compare To Constant  relop=<=  const=3  OutDataTypeStr=boolean
  Compare To Constant15 : simulink/Logic and Bit Operations/Compare To Constant  relop=<=  const=6  OutDataTypeStr=boolean
  Compare To Constant16 : simulink/Logic and Bit Operations/Compare To Constant  relop=<=  const=9  OutDataTypeStr=boolean
  Compare To Constant18 : simulink/Logic and Bit Operations/Compare To Constant  relop=<=  const=1  OutDataTypeStr=boolean
  Compare To Constant2 : simulink/Logic and Bit Operations/Compare To Constant  relop=<=  const=3  OutDataTypeStr=boolean
  Compare To Constant4 : simulink/Logic and Bit Operations/Compare To Constant  relop=<=  const=3  OutDataTypeStr=boolean
  Compare To Constant7 : simulink/Logic and Bit Operations/Compare To Constant  relop=<=  const=0.32  OutDataTypeStr=boolean
  Compare To Constant9 : simulink/Logic and Bit Operations/Compare To Constant  relop=<=  const=1.2  OutDataTypeStr=boolean
  Constant1 : Constant
  Constant10 : Constant  Value=0
  Constant11 : Constant  Value=0.7
  Constant12 : Constant  Value=0.95
  Constant13 : Constant  Value=4
  Constant14 : Constant  Value=1.05
  Constant15 : Constant  Value=0
  Constant16 : Constant  Value=1.1
  Constant17 : Constant  Value=27
  Constant18 : Constant  Value=1.2
  Constant19 : Constant  Value=26
  Constant2 : Constant  Value=0.7
  Constant3 : Constant  Value=0.5
  Constant4 : Constant  Value=0.25
  Constant5 : Constant  Value=8
  Constant6 : Constant  Value=11
  Constant7 : Constant  Value=12
  Constant8 : Constant  Value=14
  Constant9 : Constant  Value=18
  OR{1..9} (9 alike) : Logic  IconShape=distinctive  AllPortsSameDT=off  OutDataTypeStr=boolean
  Sum{1..10} (10 alike) : Sum  Inputs=|+-
  Switch{1..9} (9 alike) : Switch  Criteria=u2 > Threshold
  Vpu : Outport  VectorParamsAs1DForOutWhenUnconnected=on
  wires:
  Constant2/1 -> Switch2/1
  Switch2/1 -> Switch1/3
  Switch9/1 -> Switch2/3
  OR7/1 -> Switch1/2
  Constant3/1 -> Switch1/1
  OR8/1 -> Switch2/2
  Sum4/1 -> Compare To Constant10/1, Compare To Constant11/1
  Constant5/1 -> Sum4/2
  OR6/1 -> Switch5/2
  Compare To Constant10/1 -> OR6/1
  Compare To Constant11/1 -> OR6/2
  Compare To Constant7/1 -> OR1/2
  Compare To Constant6/1 -> OR1/1
  Constant6/1 -> Sum1/2
  Sum1/1 -> Compare To Constant7/1, Compare To Constant6/1
  Sum2/1 -> Compare To Constant8/1, Compare To Constant9/1
  Constant7/1 -> Sum2/2
  Compare To Constant8/1 -> OR5/1
  Compare To Constant9/1 -> OR5/2
  Compare To Constant13/1 -> OR7/2
  Compare To Constant12/1 -> OR7/1
  Constant8/1 -> Sum3/2
  Sum3/1 -> Compare To Constant13/1, Compare To Constant12/1
  Sum5/1 -> Compare To Constant14/1, Compare To Constant15/1
  Constant9/1 -> Sum5/2
  Compare To Constant14/1 -> OR8/1
  Compare To Constant15/1 -> OR8/2
  Constant4/1 -> Switch3/1
  OR5/1 -> Switch3/2
  OR1/1 -> Switch4/2
  Constant10/1 -> Switch4/1
  Constant11/1 -> Switch5/1
  Switch1/1 -> Switch3/3
  Switch3/1 -> Switch4/3
  Switch4/1 -> Switch5/3
  Switch5/1 -> Switch6/3
  Constant12/1 -> Switch6/1
  Compare To Constant2/1 -> OR2/2
  Compare To Constant1/1 -> OR2/1
  OR2/1 -> Switch6/2
  Constant13/1 -> Sum6/2
  Sum6/1 -> Compare To Constant2/1, Compare To Constant1/1
  Sum7/1 -> Compare To Constant3/1, Compare To Constant4/1
  Constant15/1 -> Sum7/2
  OR3/1 -> Switch7/2
  Compare To Constant3/1 -> OR3/1
  Compare To Constant4/1 -> OR3/2
  Constant14/1 -> Switch7/1
  Switch6/1 -> Switch7/3
  Switch7/1 -> Vpu/1
  Switch8/1 -> Switch9/3
  Constant18/1 -> Switch9/1
  Sum10/1 -> Sum4/1, Sum1/1, Sum2/1, Sum3/1, Sum5/1, Sum8/1, Sum9/1, Sum6/1, Sum7/1
  Compare To Constant18/1 -> OR9/2
  Compare To Constant17/1 -> OR9/1
  OR9/1 -> Switch9/2
  Constant19/1 -> Sum9/2
  Sum9/1 -> Compare To Constant18/1, Compare To Constant17/1
  Sum8/1 -> Compare To Constant5/1, Compare To Constant16/1
  Constant17/1 -> Sum8/2
  OR4/1 -> Switch8/2
  Compare To Constant5/1 -> OR4/1
  Compare To Constant16/1 -> OR4/2
  Constant16/1 -> Switch8/1
  Constant1/1 -> Switch8/3
  Clock1/1 -> Sum10/1
  StartTime/1 -> Sum10/2

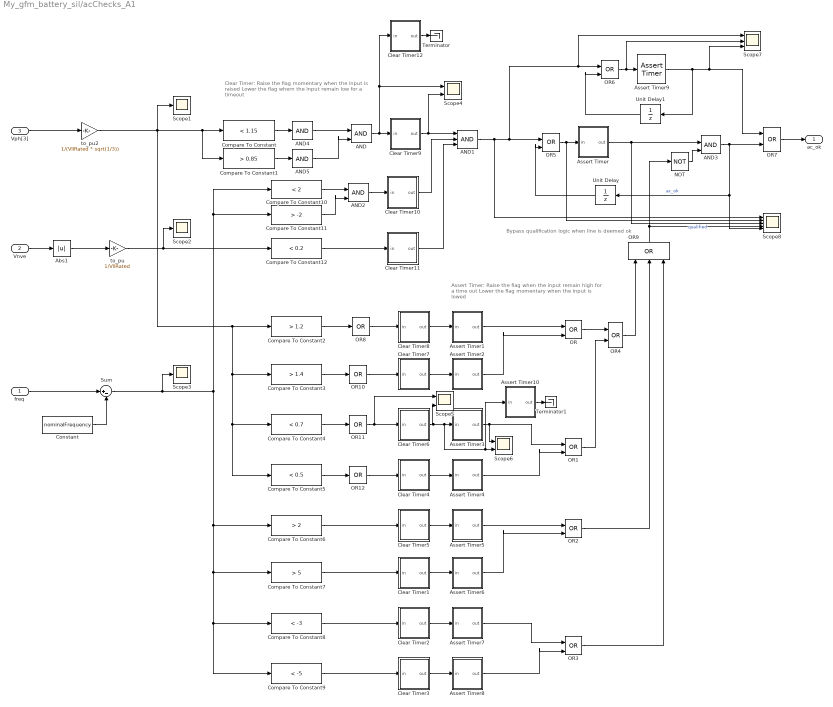
== system My_gfm_battery_sil/acChecks_A1 ==
  note: Clear Timer:
      | Raise the flag momentary when the input is raised
      | Lower the flag whern the input remain low for a timeout
  note: Bypass qualification logic when line is deemed ok
  note: Assert Timer:
      | Raise the flag when the input remain high for a time out
      | Lower the flag momentary when the input is lowed
  freq : Inport
  Vnve : Inport  Port=2
  Vph[3] : Inport  Port=3
  AND : Logic  IconShape=distinctive  AllPortsSameDT=off  OutDataTypeStr=boolean
  AND1 : Logic  Inputs=3  IconShape=distinctive  AllPortsSameDT=off  OutDataTypeStr=boolean
  AND2 : Logic  IconShape=distinctive  AllPortsSameDT=off  OutDataTypeStr=boolean
  AND3 : Logic  IconShape=distinctive  AllPortsSameDT=off  OutDataTypeStr=boolean
  AND4 : Logic  Inputs=1  IconShape=distinctive  AllPortsSameDT=off  OutDataTypeStr=boolean
  AND5 : Logic  Inputs=1  IconShape=distinctive  AllPortsSameDT=off  OutDataTypeStr=boolean
  Abs1 : Abs
  Assert Timer : Subsystem  mask{T_STEP=T_CNTL, TIMEOUT=300}
      mask prompts: T_STEP "Time step"
  Assert Timer1 : Subsystem  mask{T_STEP=T_CNTL, TIMEOUT=60}
      mask prompts: T_STEP "Time step"
  Assert Timer10 : Subsystem  mask{T_STEP=T_CNTL, TIMEOUT=60}
      mask prompts: T_STEP "Time step"
  Assert Timer2 : Subsystem  mask{T_STEP=T_CNTL, TIMEOUT=10}
      mask prompts: T_STEP "Time step"
  Assert Timer3 : Subsystem  mask{T_STEP=T_CNTL, TIMEOUT=60}
      mask prompts: T_STEP "Time step"
  Assert Timer4 : Subsystem  mask{T_STEP=T_CNTL, TIMEOUT=10}
      mask prompts: T_STEP "Time step"
  Assert Timer5 : Subsystem  mask{T_STEP=T_CNTL, TIMEOUT=60}
      mask prompts: T_STEP "Time step"
  Assert Timer6 : Subsystem  mask{T_STEP=T_CNTL, TIMEOUT=10}
      mask prompts: T_STEP "Time step"
  Assert Timer7 : Subsystem  mask{T_STEP=T_CNTL, TIMEOUT=60}
      mask prompts: T_STEP "Time step"
  Assert Timer8 : Subsystem  mask{T_STEP=T_CNTL, TIMEOUT=10}
      mask prompts: T_STEP "Time step"
  Assert Timer9 : controls_element_lib/acChecks_A/Assert Timer  T_STEP=T_CNTL  TIMEOUT=tRequalify
  Clear Timer1 : Subsystem  mask{T_STEP=T_CNTL, TIMEOUT=0.1, TIMER_INIT=0.1}
      mask prompts: T_STEP "Time step"; TIMER_INIT "Timer initial value"
  Clear Timer10 : Subsystem  mask{T_STEP=T_CNTL, TIMEOUT=0.1, TIMER_INIT=0}
      mask prompts: T_STEP "Time step"; TIMER_INIT "Timer initial value"
  Clear Timer11 : Subsystem  mask{T_STEP=T_CNTL, TIMEOUT=0.1, TIMER_INIT=0}
      mask prompts: T_STEP "Time step"; TIMER_INIT "Timer initial value"
  Clear Timer12 : Subsystem  mask{T_STEP=T_CNTL, TIMEOUT=0.1, TIMER_INIT=0}
      mask prompts: T_STEP "Time step"; TIMER_INIT "Timer initial value"
  Clear Timer2 : Subsystem  mask{T_STEP=T_CNTL, TIMEOUT=0.1, TIMER_INIT=0.1}
      mask prompts: T_STEP "Time step"; TIMER_INIT "Timer initial value"
  Clear Timer3 : Subsystem  mask{T_STEP=T_CNTL, TIMEOUT=0.1, TIMER_INIT=0.1}
      mask prompts: T_STEP "Time step"; TIMER_INIT "Timer initial value"
  Clear Timer4 : Subsystem  mask{T_STEP=T_CNTL, TIMEOUT=0.1, TIMER_INIT=0}
      mask prompts: T_STEP "Time step"; TIMER_INIT "Timer initial value"
  Clear Timer5 : Subsystem  mask{T_STEP=T_CNTL, TIMEOUT=0.1, TIMER_INIT=0.1}
      mask prompts: T_STEP "Time step"; TIMER_INIT "Timer initial value"
  Clear Timer6 : Subsystem  mask{T_STEP=T_CNTL, TIMEOUT=0.1, TIMER_INIT=0}
      mask prompts: T_STEP "Time step"; TIMER_INIT "Timer initial value"
  Clear Timer7 : Subsystem  mask{T_STEP=T_CNTL, TIMEOUT=0.1, TIMER_INIT=0}
      mask prompts: T_STEP "Time step"; TIMER_INIT "Timer initial value"
  Clear Timer8 : Subsystem  mask{T_STEP=T_CNTL, TIMEOUT=0.1, TIMER_INIT=0}
      mask prompts: T_STEP "Time step"; TIMER_INIT "Timer initial value"
  Clear Timer9 : Subsystem  mask{T_STEP=T_CNTL, TIMEOUT=0.1, TIMER_INIT=0}
      mask prompts: T_STEP "Time step"; TIMER_INIT "Timer initial value"
  Compare To Constant : simulink/Logic and Bit Operations/Compare To Constant  relop=<  const=1.15  OutDataTypeStr=boolean
  Compare To Constant1 : simulink/Logic and Bit Operations/Compare To Constant  relop=>  const=0.85  OutDataTypeStr=boolean
  Compare To Constant10 : simulink/Logic and Bit Operations/Compare To Constant  relop=<  const=2  OutDataTypeStr=boolean
  Compare To Constant11 : simulink/Logic and Bit Operations/Compare To Constant  relop=>  const=-2  OutDataTypeStr=boolean
  Compare To Constant12 : simulink/Logic and Bit Operations/Compare To Constant  relop=<  const=0.2  OutDataTypeStr=boolean
  Compare To Constant2 : simulink/Logic and Bit Operations/Compare To Constant  relop=>  const=1.2  OutDataTypeStr=boolean
  Compare To Constant3 : simulink/Logic and Bit Operations/Compare To Constant  relop=>  const=1.4  OutDataTypeStr=boolean
  Compare To Constant4 : simulink/Logic and Bit Operations/Compare To Constant  relop=<  const=0.7  OutDataTypeStr=boolean
  Compare To Constant5 : simulink/Logic and Bit Operations/Compare To Constant  relop=<  const=0.5  OutDataTypeStr=boolean
  Compare To Constant6 : simulink/Logic and Bit Operations/Compare To Constant  relop=>  const=2  OutDataTypeStr=boolean
  Compare To Constant7 : simulink/Logic and Bit Operations/Compare To Constant  relop=>  const=5  OutDataTypeStr=boolean
  Compare To Constant8 : simulink/Logic and Bit Operations/Compare To Constant  relop=<  const=-3  OutDataTypeStr=boolean
  Compare To Constant9 : simulink/Logic and Bit Operations/Compare To Constant  relop=<  const=-5  OutDataTypeStr=boolean
  Constant : Constant  Value=nominalFrequency
  NOT : Logic  Operator=NOT  IconShape=distinctive  AllPortsSameDT=off  OutDataTypeStr=boolean
  OR{,1..7} (8 alike) : Logic  Operator=OR  IconShape=distinctive  AllPortsSameDT=off  OutDataTypeStr=boolean
  OR{8,10..12} (4 alike) : Logic  Operator=OR  Inputs=1  IconShape=distinctive  AllPortsSameDT=off  OutDataTypeStr=boolean
  OR9 : Logic  Operator=OR  Inputs=3  IconShape=distinctive  AllPortsSameDT=off  OutDataTypeStr=boolean
  Scope1 : Scope
  Scope2 : Scope
  Scope3 : Scope
  Scope4 : Scope  NumInputPorts=2
  Scope5 : Scope  NumInputPorts=2
  Scope6 : Scope  NumInputPorts=2
  Scope7 : Scope  NumInputPorts=3
  Scope8 : Scope  NumInputPorts=5
  Sum : Sum  Inputs=|+-
  Terminator : Terminator
  Terminator1 : Terminator
  Unit Delay : UnitDelay  SampleTime=T_CNTL
  Unit Delay1 : UnitDelay  SampleTime=T_CNTL
  to_pu : Gain  Gain=1/VllRated
  to_pu2 : Gain  Gain=1/(VllRated * sqrt(1/3))
  ac_ok : Outport  VectorParamsAs1DForOutWhenUnconnected=on
  wires:
  Vph[3]/1 -> to_pu2/1
  OR4/1 -> OR9/1
  OR9/1 -> NOT/1, Scope8/4
  OR7/1 -> ac_ok/1
  Assert Timer9/1 -> Unit Delay1/1, Scope7/3, OR7/1
  OR6/1 -> Scope7/2, Assert Timer9/1
  Unit Delay1/1 -> OR6/2
  Constant/1 -> Sum/2
  freq/1 -> Sum/1
  to_pu/1 -> Scope2/1, Compare To Constant12/1
  to_pu2/1 -> Scope1/1, Compare To Constant/1, Compare To Constant1/1, Compare To Constant2/1, Compare To Constant5/1, Compare To Constant4/1, Compare To Constant3/1
  Abs1/1 -> to_pu/1
  Unit Delay/1 -> OR5/2
  Assert Timer1/1(out) -> OR/1
  Compare To Constant12/1 -> Clear Timer11/1(in)
  Clear Timer11/1(out) -> AND1/3
  Compare To Constant2/1 -> OR8/1
  Compare To Constant1/1 -> AND5/1
  Assert Timer/1(out) -> AND3/1, Scope8/3  "qualified"
  OR3/1 -> OR9/3
  Assert Timer4/1(out) -> OR1/2
  Assert Timer5/1(out) -> OR2/1
  Clear Timer5/1(out) -> Assert Timer5/1(in)
  Compare To Constant6/1 -> Clear Timer5/1(in)
  Clear Timer1/1(out) -> Assert Timer6/1(in)
  Clear Timer8/1(out) -> Assert Timer1/1(in)
  Assert Timer7/1(out) -> OR3/1
  Assert Timer8/1(out) -> OR3/2
  Vnve/1 -> Abs1/1
  NOT/1 -> AND3/2
  Assert Timer3/1(out) -> Scope6/1, OR1/1
  Compare To Constant/1 -> AND4/1
  Compare To Constant3/1 -> OR10/1
  AND2/1 -> Clear Timer10/1(in)
  Compare To Constant9/1 -> Clear Timer3/1(in)
  Compare To Constant11/1 -> AND2/2
  Compare To Constant4/1 -> OR11/1
  Assert Timer6/1(out) -> OR2/2
  Clear Timer6/1(out) -> Scope5/2, Assert Timer10/1(in), Scope6/2, Assert Timer3/1(in)
  Compare To Constant8/1 -> Clear Timer2/1(in)
  OR1/1 -> OR4/2
  Clear Timer2/1(out) -> Assert Timer7/1(in)
  Compare To Constant5/1 -> OR12/1
  Compare To Constant7/1 -> Clear Timer1/1(in)
  Clear Timer10/1(out) -> AND1/2
  Clear Timer3/1(out) -> Assert Timer8/1(in)
  Clear Timer7/1(out) -> Assert Timer2/1(in)
  Sum/1 -> Scope3/1, Compare To Constant11/1, Compare To Constant10/1, Compare To Constant6/1, Compare To Constant7/1, Compare To Constant8/1, Compare To Constant9/1
  Assert Timer2/1(out) -> OR/2
  Compare To Constant10/1 -> AND2/1
  Clear Timer9/1(out) -> Scope4/2, AND1/1
  OR/1 -> OR4/1
  Clear Timer4/1(out) -> Assert Timer4/1(in)
  AND3/1 -> Scope8/5, Unit Delay/1, OR7/2  "ac_ok"
  OR2/1 -> OR9/2
  OR8/1 -> Clear Timer8/1(in)
  OR10/1 -> Clear Timer7/1(in)
  OR11/1 -> Clear Timer6/1(in), Scope5/1
  OR12/1 -> Clear Timer4/1(in)
  AND/1 -> Clear Timer12/1(in), Scope4/1, Clear Timer9/1(in)
  AND4/1 -> AND/1
  AND5/1 -> AND/2
  Clear Timer12/1(out) -> Terminator/1
  Assert Timer10/1(out) -> Terminator1/1
  AND1/1 -> OR5/1, Scope7/1, OR6/1, Scope8/1
  OR5/1 -> Scope8/2, Assert Timer/1(in)

== system My_gfm_battery_sil/acMonitor_A  ==
  note: RMS LL Pos Seq Voltage (Vd+, Vq+)
  note: RMS LL Neg Seq Voltage (Vd-, Vq-)
  note: cos x + j sin x
      | cos (x-120) + j (sin x -120)
      | cos (x+120) + j (sin x +120)
  note: Hz
  note: RMS Va, Vb, Vc
  v_ac : Inport
  Analyzer_V : Subsystem
  Analyzer_V1 : Subsystem  Commented=on
  Gain2 : Gain  Gain=2
  PLL_3ph : Subsystem
  RMS_Analyzer : Subsystem
  SOGI : Subsystem
  Scope : Scope  NumInputPorts=3
  Scope1 : Scope  NumInputPorts=4
  Terminator : Terminator
  to_pu : Gain  Gain=1/VllRated
  pll_freq : Outport  VectorParamsAs1DForOutWhenUnconnected=on
  pll_osc[3] : Outport  Port=2  VectorParamsAs1DForOutWhenUnconnected=on
  Vpve : Outport  Port=3  VectorParamsAs1DForOutWhenUnconnected=on
  Vnve : Outport  Port=4  VectorParamsAs1DForOutWhenUnconnected=on
  Vph[3] : Outport  Port=5  VectorParamsAs1DForOutWhenUnconnected=on
  wires:
  SOGI/1(notch) -> Scope/3, Vph[3]/1
  Gain2/1 -> SOGI/2(fnom)
  RMS_Analyzer/1(RMS) -> Scope/2, SOGI/1(in)
  Analyzer_V/4(Nve) -> Scope1/4, Vnve/1
  Analyzer_V/3(Pve) -> Vpve/1, Scope1/3
  PLL_3ph/1(osc[3]) -> pll_osc[3]/1, Analyzer_V/2(osc[3])
  PLL_3ph/2(freq) -> Gain2/1, pll_freq/1
  v_ac/1 -> to_pu/1, Analyzer_V/1(in[3]), Scope/1, RMS_Analyzer/1(in)
  to_pu/1 -> PLL_3ph/1(ref)
  Analyzer_V/1(fund[3]) -> Scope1/1
  Analyzer_V/2(Zero) -> Scope1/2
  SOGI/2(bpf) -> Terminator/1

== system My_gfm_battery_sil/currentLimiting_B ==
  note: SOGI gain is 1 not 1/sqrt(2),
      | improve tracking over transients
  note: Only capture 60Hz component
  note: Iabc rms
  note: Peak_Iabc
  note: Only apply limit on 60 Hz components
  Irms_limit : Inport
  freq : Inport  Port=2
  iref : Inport  Port=3
  Product1 : Product
  RMS_Analyzer : Subsystem
  SOGI_BPF : Subsystem
  Scope11 : Scope  NumInputPorts=3
  Sum1 : Sum  Inputs=|+-
  estimate_excess : Subsystem
  soft_saturation : Subsystem  mask{soft_limit=peakSoftLimit*IRated, hard_limit=peakHardLimit*IRated, Xau=1}
      mask prompts: soft_limit "Soft limit"; hard_limit "Hard limit"; Xau "Saturation Rate"
  soft_saturation1 : Subsystem  Commented=on  mask{soft_limit=peakSoftLimit*IRated, hard_limit=peakHardLimit*IRated}
      mask prompts: soft_limit "Soft limit"; hard_limit "Hard limit"
  iref_limited : Outport  VectorParamsAs1DForOutWhenUnconnected=on
  wires:
  soft_saturation/1(out) -> iref_limited/1
  estimate_excess/1(excess_fraction) -> Scope11/1, Product1/1
  RMS_Analyzer/1(RMS) -> estimate_excess/2(I[3])  "Irms"
  Product1/1 -> Scope11/3, Sum1/2  "i_excess"
  Sum1/1 -> soft_saturation/1(in)
  SOGI_BPF/1(bpf) -> Product1/2, Scope11/2
  freq/1 -> SOGI_BPF/2(f)
  iref/1 -> Sum1/1, RMS_Analyzer/1(in), SOGI_BPF/1(in)
  Irms_limit/1 -> estimate_excess/1(Ilimit)

== system My_gfm_battery_sil/phasor_analysis3 ==
  v : Inport
  osc : Inport  Port=2
  Complex to Magnitude-Angle : ComplexToMagnitudeAngle
  Complex to Real-Imag : ComplexToRealImag
  Conj : Math  Operator=conj  SaturateOnIntegerOverflow=on
  Gain : Gain  Gain=sqrt(2)
  Gain1 : Gain  Gain=1/3
  Gain2 : Gain  Gain=sqrt(3)
  Product3 : Product
  Real-Imag to Complex : RealImagToComplex
  Scope : Scope  NumInputPorts=4
  Sum of Elements1 : Sum  Inputs=+
  Transfer Fcn : TransferFcn  Denominator=[0.01 1]
  Transfer Fcn1 : TransferFcn  Denominator=[0.01 1]
  magnitude : Outport  VectorParamsAs1DForOutWhenUnconnected=on
  phase : Outport  Port=2  VectorParamsAs1DForOutWhenUnconnected=on
  wires:
  Complex to Magnitude-Angle/2 -> phase/1
  Complex to Magnitude-Angle/1 -> magnitude/1
  Gain2/1 -> Complex to Magnitude-Angle/1
  Gain1/1 -> Complex to Real-Imag/1
  Gain/1 -> Scope/2, Product3/2
  Real-Imag to Complex/1 -> Gain2/1
  Conj/1 -> Gain/1
  osc/1 -> Conj/1
  Complex to Real-Imag/1 -> Transfer Fcn/1
  v/1 -> Scope/1, Product3/1
  Complex to Real-Imag/2 -> Transfer Fcn1/1
  Product3/1 -> Scope/3, Sum of Elements1/1
  Transfer Fcn/1 -> Real-Imag to Complex/1
  Sum of Elements1/1 -> Scope/4, Gain1/1
  Transfer Fcn1/1 -> Real-Imag to Complex/2

== system My_gfm_battery_sil/soft_saturation ==
  note: 1-e(-dx/H)
  note: dX
  note: dX/Xau
  note: -1+e(-dx/H)
  note: H*[1-e(-dx/H)] + H*[-1+e(-dx/H)]
  in : Inport
  Constant : Constant
  Constant1 : Constant
  Exp : Math  SaturateOnIntegerOverflow=on
  Exp1 : Math  SaturateOnIntegerOverflow=on
  Gain : Gain  Gain=-1
  Gain1 : Gain  Gain=Xau
  Product : Product  Inputs=*/
  Sum : Sum  Inputs=|++
  Sum1 : Sum  Inputs=-+|
  Sum2 : Sum  Inputs=|+-
  Sum3 : Sum  Inputs=|+-
  Sum4 : Sum  Inputs=|++
  headroom : Gain  Gain=(hard_limit - soft_limit)
  headroom1 : Constant  Value=max(hard_limit - soft_limit, 1e-3)
  negative : Saturate  UpperLimit=0  LowerLimit=-inf
  positive : Saturate  UpperLimit=inf  LowerLimit=0
  soft_limit : Saturate  UpperLimit=soft_limit  LowerLimit=-soft_limit
  out : Outport  VectorParamsAs1DForOutWhenUnconnected=on
  wires:
  headroom1/1 -> Gain1/1
  Sum1/1 -> Product/1
  Sum2/1 -> Sum4/1
  Sum4/1 -> headroom/1
  Gain/1 -> Exp/1
  headroom/1 -> Sum/2
  Exp/1 -> Sum2/2
  positive/1 -> Gain/1
  in/1 -> soft_limit/1, Sum1/2
  Exp1/1 -> Sum3/1
  Sum/1 -> out/1
  soft_limit/1 -> Sum1/1, Sum/1
  Sum3/1 -> Sum4/2
  negative/1 -> Exp1/1
  Constant1/1 -> Sum3/2
  Product/1 -> positive/1, negative/1
  Constant/1 -> Sum2/1
  Gain1/1 -> Product/2  "Xau"

== system My_gfm_battery_sil/step-sequence ==
  StartTime : Inport
  Clock1 : Clock
  Compare To Constant1 : simulink/Logic and Bit Operations/Compare To Constant  relop=>  const=0  OutDataTypeStr=boolean
  Compare To Constant2 : simulink/Logic and Bit Operations/Compare To Constant  relop=<=  const=100  OutDataTypeStr=boolean
  Compare To Constant3 : simulink/Logic and Bit Operations/Compare To Constant  relop=>  const=0  OutDataTypeStr=boolean
  Compare To Constant4 : simulink/Logic and Bit Operations/Compare To Constant  relop=<=  const=3  OutDataTypeStr=boolean
  Constant1 : Constant
  Constant12 : Constant  Value=0.6
  Constant13 : Constant  Value=5
  Constant14 : Constant  Value=0.8
  Constant15 : Constant  Value=0
  OR2 : Logic  IconShape=distinctive  AllPortsSameDT=off  OutDataTypeStr=boolean
  OR3 : Logic  IconShape=distinctive  AllPortsSameDT=off  OutDataTypeStr=boolean
  Sum10 : Sum  Inputs=|+-
  Sum6 : Sum  Inputs=|+-
  Sum7 : Sum  Inputs=|+-
  Switch6 : Switch  Criteria=u2 > Threshold
  Switch7 : Switch  Criteria=u2 > Threshold
  pu : Outport  VectorParamsAs1DForOutWhenUnconnected=on
  wires:
  Constant12/1 -> Switch6/1
  Compare To Constant2/1 -> OR2/2
  Compare To Constant1/1 -> OR2/1
  OR2/1 -> Switch6/2
  Constant13/1 -> Sum6/2
  Sum6/1 -> Compare To Constant2/1, Compare To Constant1/1
  Sum7/1 -> Compare To Constant3/1, Compare To Constant4/1
  Constant15/1 -> Sum7/2
  OR3/1 -> Switch7/2
  Compare To Constant3/1 -> OR3/1
  Compare To Constant4/1 -> OR3/2
  Constant14/1 -> Switch7/1
  Switch6/1 -> Switch7/3
  Switch7/1 -> pu/1
  Sum10/1 -> Sum6/1, Sum7/1
  Clock1/1 -> Sum10/1
  StartTime/1 -> Sum10/2
  Constant1/1 -> Switch6/3
